simulink model "Detumbling"  (R2024b)
settings: Solver=ode4  StartTime=0.0  StopTime=2000  FixedStep=0.1  RelTol=1e-3
values from neighbouring files (symbols this model uses):
  A = A + DCM_out_slew(:,:,jj)    [sadcode.m]
  a = 6899750    [sadcode.m]
  Area_vect = [3;3;3;3;1;1;1;1;1;1]    [sadcode.m]
  C_d = 2.2    [sadcode.m]
  e = 0.0005895    [sadcode.m]
  G = 6.67e-11    [sadcode.m]
  g = [g1_0 g2_0 g3_0 g4_0 g5_0 g6_0 g7_0 g8_0 g9_0 g10_0  g11_0  g12_0  g13_0 ... (first row only)    [IGRF13.m]
  h = [h1_0 h2_0 h3_0 h4_0 h5_0 h6_0 h7_0 h8_0 h9_0 h10_0  h11_0  h12_0  h13_0 ... (first row only)    [IGRF13.m]
  I = diag([Ix,Iy,Iz])    [sadcode.m]
  i = deg2rad(5.0097)    [sadcode.m]
  Ix = 4.208e11*10^(-3-6)    (= 420.8)    [sadcode.m]
  Iy = 4.922e12*10^(-3-6)    (= 4922)    [sadcode.m]
  Iz = 4.399e12*10^(-3-6)    (= 4399)    [sadcode.m]
  J_b = [1 ; 18 ; 5]    [sadcode.m]
  k_det = 110    [sadcode.m]
  M = 5.97219e24    (= 5.97219e+24)    [sadcode.m]
  Mount = [0 0 1 0 1 0]    [sadcode.m]
  mu = G*M    (= 398345073000000)    [sadcode.m]
  n = sqrt(mu/a^3)    [sadcode.m]
  N_b = [0,0,+1; 0,0,-1; 0,0,1; 0,0,-1;1,0,0 ; -1,0,0; 0,1,0; 0,-1,0; 0,0,1; 0,0,-1]    [sadcode.m]
  n_face = length(rho_s)    [sadcode.m]
  p = a * (1 - e^2)    (= 6899747.60227)    [sadcode.m]
  q = abs(q(:,1))    [sadcode.m]
  R_f = [2.5,0,0; 2.5,0,0; -2.5,0,0; -2.5,0,0; 1,0,0; -1,0,0; 0,1,0; 0,-1,0; 0,0,1; 0,0,-1]    [sadcode.m]
  R_sun = 149597870700    [sadcode.m]
  rho = 3.13e-13    [sadcode.m]
  theta0 = theta0_slew(jj)    [sadcode.m]
  w0x = w_out_slew(1,jj)    [sadcode.m]
  w0y = w_out_slew(2,jj)    [sadcode.m]
  w0z = w_out_slew(3,jj)    [sadcode.m]
  w_earth = 2*pi/(24*3600)    (= 7.27220521664e-05)    [sadcode.m]
undefined symbols (not defined in the file or in its folder): DiscIntNeverNeededParam
libraries: matrix_library x6, simulink x5
settings Model: Creator=andre  LastModifiedBy=andre
settings OptimizationCC: ReuseModelBlockBuffer=off
settings RTWCC: GPUComputeCapability=3.5

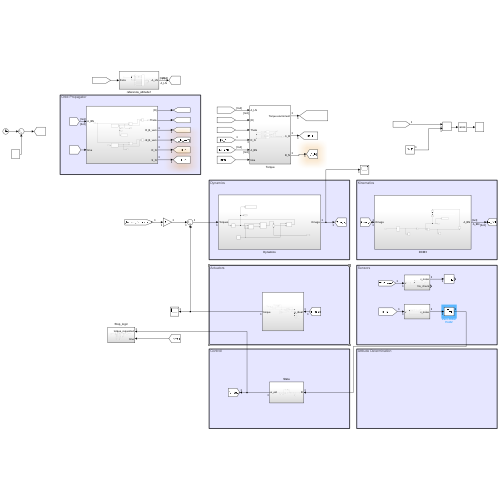
[thumbnail: Simulink's stored preview of the top-level diagram]
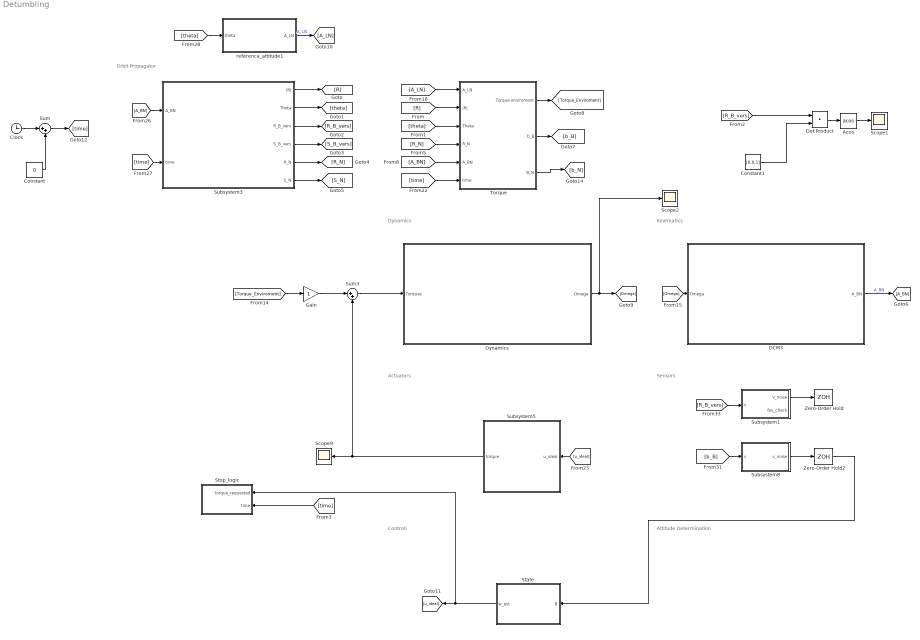
== system Detumbling ==
  note: Orbit Propagator
  note: Dynamics
  note: Kinematics
  note: Sensors
  note: Attitude Determination
  note: Controll
  note: Actuators
  Acos : Trigonometry  Operator=acos
  Clock : Clock
  Constant : Constant  Value=0
  Constant1 : Constant  Value=[0,0,1]
  DCM3 : Subsystem
  Dot Product : DotProduct  OutDataTypeStr=Inherit: Inherit via internal rule
  Dynamics : Subsystem
  Gain : Gain
  Scope1 : Scope
  Scope2 : Scope
  Scope9 : Scope
  State : Subsystem
  Stop_logic : Subsystem
  Subsystem1 : Subsystem
  Subsystem3 : Subsystem
  Subsystem5 : Subsystem
  Subsystem8 : Subsystem
  Sum : Sum  Inputs=|++
  Sum3 : Sum  Inputs=|++
  Torque : Subsystem
  Zero-Order Hold : ZeroOrderHold
  Zero-Order Hold2 : ZeroOrderHold  SampleTime=0.1
  referenca_attitude1 : Subsystem
  wires:
  Sum3/1 -> Dynamics/1(Torques)
  Subsystem5/1(torque) -> Scope9/1, Sum3/2
  Subsystem3/2(Theta) -> [theta]
  Subsystem3/3(R_B_vers) -> [R_B_vers]
  Subsystem3/4(S_B_vers) -> [S_B_vers]
  Subsystem3/5(R_N) -> [R_N]
  Subsystem3/6(S_N) -> [S_N]
  DCM3/1(A_BN) -> [A_BN]  "A_BN"
  [Torque_Enviroment] -> Gain/1
  Dynamics/1(Omega) -> Scope2/1, [Omega]
  [Omega] -> DCM3/1(Omega)
  referenca_attitude1/1(A_LN) -> [A_LN]  "A_LN"
  [theta] -> referenca_attitude1/1(theta)
  [u_ideal] -> Subsystem5/1(u_ideal)
  Subsystem3/1(|R|) -> [R]
  Clock/1 -> Sum/1
  Constant/1 -> Sum/2
  Sum/1 -> [time]
  [A_BN] -> Subsystem3/1(A_BN)
  [time] -> Subsystem3/2(time)
  State/1(w_est) -> Stop_logic/1(torque_requested), [u_ideal]
  [b_B] -> Subsystem8/1(v)
  [R_B_vers] -> Subsystem1/1(v)
  Subsystem8/1(v_noise) -> Zero-Order Hold2/1
  Subsystem1/1(v_noise) -> Zero-Order Hold/1
  Zero-Order Hold2/1 -> State/1(B)
  Gain/1 -> Sum3/1
  [R_B_vers] -> Dot Product/1
  Constant1/1 -> Dot Product/2
  Dot Product/1 -> Acos/1
  Acos/1 -> Scope1/1
  [time] -> Stop_logic/2(time)
  [A_LN] -> Torque/1(A_LN)
  [R_N] -> Torque/4(R_N)
  [A_BN] -> Torque/5(A_BN)
  [time] -> Torque/6(time)
  [R] -> Torque/2(|R|)
  [theta] -> Torque/3(Theta)
  Torque/1(Torque enviroment) -> [Torque_Enviroment]
  Torque/3(B_N) -> [b_N]
  Torque/2(b_B) -> [b_B]

== system Detumbling/DCM3 ==
  note: YOU CAN ORTHORNORMALIZE MORE TIMES
  Omega : Inport
  Gain : Gain  Gain=-1
  Integrator3 : Integrator  InitialCondition=A
  ORTHONORMALIZE1 : Subsystem
  ORTHONORMALIZE3 : Subsystem
  Product3 : Product  Multiplication=Matrix(*)
  Scope : Scope
  Scope2 : Scope
  To Workspace1 : ToWorkspace  VariableName=real_DCM_det  SampleTime=-1
  w->w^ : Subsystem
  A_BN : Outport
  wires:
  Gain/1 -> Product3/1
  Omega/1 -> w->w^/1(In1)
  w->w^/1(Out1) -> Gain/1, Scope/1
  Product3/1 -> Integrator3/1, Scope2/1
  Integrator3/1 -> ORTHONORMALIZE1/1(In1)
  ORTHONORMALIZE1/1(u) -> ORTHONORMALIZE3/1(In1)
  ORTHONORMALIZE3/1(u) -> To Workspace1/1, A_BN/1, Product3/2

== system Detumbling/Dynamics ==
  Torques : Inport
  Constant : Constant  Value=I
  Cross Product : matrix_library/Cross Product
  Integrator : Integrator  InitialCondition=[w0x;w0y;w0z]
  Matrix Multiply2 : Product  Inputs=/*  Multiplication=Matrix(*)
  Matrix Multiply3 : Product  Inputs=**  Multiplication=Matrix(*)
  Sum1 : Sum  Inputs=-+
  To Workspace : ToWorkspace  VariableName=w_out_det  SampleTime=-1
  Omega : Outport
  wires:
  Matrix Multiply2/1 -> Integrator/1
  Matrix Multiply3/1 -> Cross Product/2
  Cross Product/1 -> Sum1/1
  Constant/1 -> Matrix Multiply2/1, Matrix Multiply3/1
  Torques/1 -> Sum1/2
  Integrator/1 -> Cross Product/1, Matrix Multiply3/2, To Workspace/1, Omega/1
  Sum1/1 -> Matrix Multiply2/2

== system Detumbling/State ==
  B : Inport
  Cross Product : matrix_library/Cross Product
  Discrete Derivative : simulink/Discrete/Discrete Derivative  gainval=1.0  ICPrevScaledInput=0.0  OutMin=[]  OutMax=[]  OutDataType=fixdt(1, 16)  OutScaling=2^-10  DoSatur=off
  Gain : Gain  Gain=k_det
  Product : Product  Inputs=/*
  Scope : Scope
  Square : Math  Operator=square
  normalize2 : Subsystem
  w_est : Outport
  wires:
  Discrete Derivative/1 -> Cross Product/2
  Cross Product/1 -> Product/2
  normalize2/2(norm) -> Square/1
  Square/1 -> Product/1
  Product/1 -> Gain/1
  B/1 -> Discrete Derivative/1, normalize2/1(vector), Cross Product/1
  Gain/1 -> Scope/1, w_est/1

== system Detumbling/Stop_logic ==
  torque_requested : Inport
  time : Inport  Port=2
  AND : Logic  IconShape=distinctive  AllPortsSameDT=off  OutDataTypeStr=boolean
  Constant2 : Constant  Value=2.5
  Constant3 : Constant  Value=100
  Integrator : Integrator
  Relational Operator : RelationalOperator  Operator=<=  OutDataTypeStr=boolean  RndMeth=Simplest  InputSameDT=off
  Relational Operator1 : RelationalOperator  Operator=>  OutDataTypeStr=boolean  RndMeth=Simplest  InputSameDT=off
  Scope2 : Scope
  Scope3 : Scope
  Stop Simulation : Stop
  Sum1 : Sum  Inputs=|+-
  Transport Delay : TransportDelay  DelayTime=10
  normalize2 : Subsystem
  wires:
  Relational Operator1/1 -> AND/1
  time/1 -> Relational Operator1/1
  AND/1 -> Stop Simulation/1
  Sum1/1 -> Scope2/1, Relational Operator/1
  Constant2/1 -> Relational Operator/2
  Constant3/1 -> Relational Operator1/2
  Integrator/1 -> Transport Delay/1, Sum1/1
  Relational Operator/1 -> Scope3/1, AND/2
  Transport Delay/1 -> Sum1/2
  normalize2/2(norm) -> Integrator/1
  torque_requested/1 -> normalize2/1(vector)

== system Detumbling/Subsystem1 ==
  v : Inport
  Constant : Constant  Value=[0,0,1]
  Cross Product : matrix_library/Cross Product
  FOV_check : Subsystem
  Product : Product
  Scope : Scope
  Scope1 : Scope
  Subsystem : Subsystem
  Subsystem3 : Subsystem
  normalize1 : Subsystem
  v_noise : Outport
  fov_check : Outport  Port=2
  wires:
  Product/1 -> v_noise/1, Scope1/1
  Cross Product/1 -> Subsystem/2(n)
  Constant/1 -> Cross Product/2
  Subsystem/1(Out1) -> Scope/1, Subsystem3/1(v)
  FOV_check/1(v_checked) -> Subsystem3/2(n), Subsystem/1(v), Cross Product/1
  FOV_check/2(fov_check) -> fov_check/1
  v/1 -> normalize1/1(vector)
  normalize1/1(vers) -> FOV_check/1(R_B_vers)
  Subsystem3/1(v_noise) -> Product/1
  normalize1/2(norm) -> Product/2

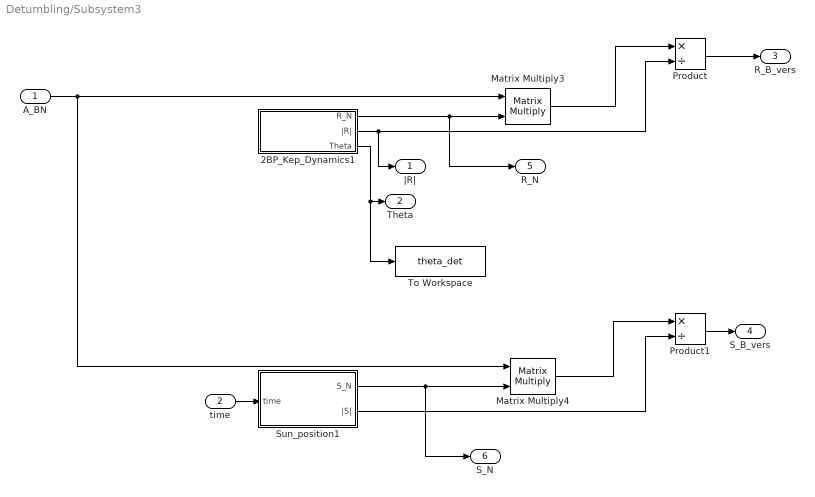
== system Detumbling/Subsystem3 ==
  A_BN : Inport
  time : Inport  Port=2
  2BP_Kep_Dynamics1 : Subsystem
  Matrix Multiply3 : Product  Multiplication=Matrix(*)
  Matrix Multiply4 : Product  Multiplication=Matrix(*)
  Product : Product  Inputs=*/
  Product1 : Product  Inputs=*/
  Sun_position1 : Subsystem
  To Workspace : ToWorkspace  VariableName=theta_det  SampleTime=-1
  |R| : Outport
  Theta : Outport  Port=2
  R_B_vers : Outport  Port=3
  S_B_vers : Outport  Port=4
  R_N : Outport  Port=5
  S_N : Outport  Port=6
  wires:
  A_BN/1 -> Matrix Multiply3/1, Matrix Multiply4/1
  2BP_Kep_Dynamics1/2(|R|) -> Product/2, |R|/1
  Matrix Multiply3/1 -> Product/1
  Matrix Multiply4/1 -> Product1/1
  2BP_Kep_Dynamics1/1(R_N) -> Matrix Multiply3/2, R_N/1
  Sun_position1/2(|S|) -> Product1/2
  Sun_position1/1(S_N) -> Matrix Multiply4/2, S_N/1
  2BP_Kep_Dynamics1/3(Theta) -> To Workspace/1, Theta/1
  Product/1 -> R_B_vers/1
  Product1/1 -> S_B_vers/1
  time/1 -> Sun_position1/1(time)

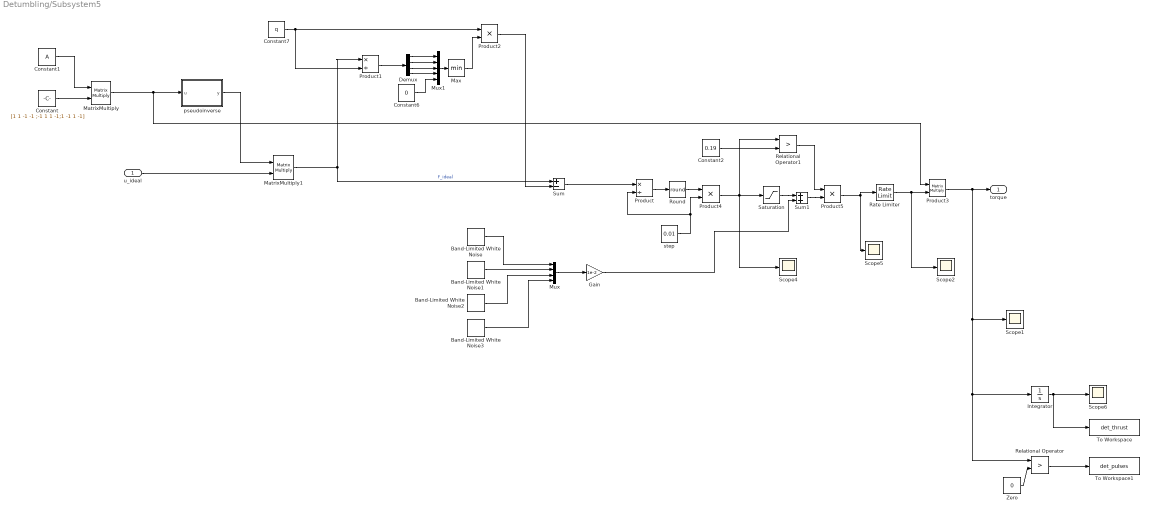
== system Detumbling/Subsystem5 ==
  u_ideal : Inport
  Band-Limited White Noise{,1..3} (4 alike) : simulink/Sources/Band-Limited White Noise  Cov=[1]  Ts=0.1  seed=[23341]
  Constant : Constant  Value=[1 1 -1 -1 ;-1 1 1 -1;1 -1 1 -1]
  Constant1 : Constant  Value=A
  Constant2 : Constant  Value=0.19
  Constant6 : Constant  Value=0
  Constant7 : Constant  Value=q
  Demux : Demux
  Gain : Gain  Gain=1e-2
  Integrator : Integrator
  MatrixMultiply : Product  Multiplication=Matrix(*)
  MatrixMultiply1 : Product  Multiplication=Matrix(*)
  Max : MinMax
  Mux : Mux
  Mux1 : Mux  Inputs=5
  Product : Product  Inputs=*/
  Product1 : Product  Inputs=*/
  Product2 : Product
  Product3 : Product  Multiplication=Matrix(*)
  Product4 : Product  Inputs=**
  Product5 : Product
  Rate Limiter : RateLimiter  RisingSlewLimit=0.5  FallingSlewLimit=-0.5  SampleTimeMode=inherited
  Relational Operator : RelationalOperator  Operator=>  OutDataTypeStr=boolean  RndMeth=Simplest  InputSameDT=off
  Relational Operator1 : RelationalOperator  Operator=>  OutDataTypeStr=boolean  RndMeth=Simplest  InputSameDT=off
  Round : Rounding  Operator=round
  Saturation : Saturate  UpperLimit=1.13  LowerLimit=0.19
  Scope{1..2,4..6} (5 alike) : Scope
  Sum : Sum  Inputs=+-
  Sum1 : Sum
  To Workspace : ToWorkspace  VariableName=det_thrust  SampleTime=-1
  To Workspace1 : ToWorkspace  VariableName=det_pulses  SampleTime=-1
  Zero : Constant  Value=0  OutDataTypeStr=Inherit: Inherit via back propagation
  pseudoinverse : MATLAB Function  TreatAsAtomicUnit=on
  step : Constant  Value=0.01
  torque : Outport
  wires:
  Band-Limited White Noise1/1 -> Mux/2
  Rate Limiter/1 -> Scope2/1, Product3/2
  Band-Limited White Noise2/1 -> Mux/3
  MatrixMultiply1/1 -> Sum/1, Product1/1  "F_ideal"
  Constant1/1 -> MatrixMultiply/1
  Mux/1 -> Gain/1
  Constant/1 -> MatrixMultiply/2
  Band-Limited White Noise/1 -> Mux/1
  Product1/1 -> Demux/1
  Band-Limited White Noise3/1 -> Mux/4
  Product2/1 -> Sum/2
  u_ideal/1 -> MatrixMultiply1/2
  pseudoinverse/1(y) -> MatrixMultiply1/1
  MatrixMultiply/1 -> Product3/1, pseudoinverse/1(u)
  Sum/1 -> Product/1
  Constant6/1 -> Mux1/5
  Constant7/1 -> Product1/2, Product2/1
  Demux/1 -> Mux1/1
  Demux/2 -> Mux1/2
  Demux/3 -> Mux1/3
  Demux/4 -> Mux1/4
  Mux1/1 -> Max/1
  Max/1 -> Product2/2
  Gain/1 -> Sum1/2
  Product5/1 -> Rate Limiter/1, Scope5/1
  Round/1 -> Product4/1
  step/1 -> Product4/2, Product/2
  Product/1 -> Round/1
  Product4/1 -> Scope4/1, Saturation/1, Relational Operator1/1
  Integrator/1 -> To Workspace/1, Scope6/1
  Zero/1 -> Relational Operator/2
  Relational Operator/1 -> To Workspace1/1
  Product3/1 -> Scope1/1, Integrator/1, Relational Operator/1, torque/1
  Relational Operator1/1 -> Product5/1
  Constant2/1 -> Relational Operator1/2
  Saturation/1 -> Sum1/1
  Sum1/1 -> Product5/2

== system Detumbling/Subsystem8 ==
  v : Inport
  Constant : Constant  Value=[0,0,1]
  Cross Product : matrix_library/Cross Product
  Product : Product
  Scope : Scope
  Scope1 : Scope
  Subsystem : Subsystem
  Subsystem3 : Subsystem
  normalize1 : Subsystem
  v_noise : Outport
  wires:
  Product/1 -> v_noise/1, Scope1/1
  Cross Product/1 -> Subsystem/2(n)
  normalize1/1(vers) -> Subsystem3/2(n), Subsystem/1(v), Cross Product/1
  Constant/1 -> Cross Product/2
  Subsystem/1(Out1) -> Scope/1, Subsystem3/1(v)
  v/1 -> normalize1/1(vector)
  Subsystem3/1(v_noise) -> Product/1
  normalize1/2(norm) -> Product/2

== system Detumbling/Torque ==
  A_LN : Inport
  |R| : Inport  Port=2
  Theta : Inport  Port=3
  R_N : Inport  Port=4
  A_BN : Inport  Port=5
  time : Inport  Port=6
  DRAG_Torque : Subsystem
  GG_Torque : Subsystem
  MAG_Torque : Subsystem
      settings: PortSchema="{\"entries\":[{\"content\":{\"sides\":[{\"content\":{\"connectorIds\":[\"In1\",\"In2\"]},\"type\":\"ConnectorPlacement.EquallySpacedRectSide\",\"uuid\":\"c54f6d6b-6c64-41b4-9c4b-666110e71804\"},{\"content\":{\"connectorIds\":[\"Out1\",\"Out2\",\"Out3\"],\"side\":\"RIGHT\"},\"type\":\"ConnectorPlacement.EquallySpacedRectSide\",\"uuid\":\"b119c4d3-4afb-4dc4-a90a-1aa1f0569df9\"},{\"content\":{\"side\":\"TOP\"},\"type\":\"ConnectorPlacement.EquallySpacedRectSide\",\"uuid\":\"da830b3a-87b4-4a36-90f7-6cd3013fb920\"},{\"content\":{\"connectorIds\":[\"In3\"],\"side\":\"BOTTOM\"},\"type\":\"ConnectorPlacement.EquallySpacedRectSide\",\"uuid\":\"c632635c-67f5-47aa-a2ed-3b005f31cd37\"}]},\"type\":\"ConnectorPlacement.EquallySpacedConnector\",\"uuid\":\"fdb04bfd-e1a8-4c42-a1d7-57e7f291fe41\"}],\"packageUris\":[\"http://schema.mathworks.com/mf0/Connector/R2020b\"],\"version\":\"1.0\"}"
  Scope : Scope
  Scope1 : Scope
  Sum : Sum  Inputs=+++
  Torque enviroment : Outport
  b_B : Outport  Port=2
  B_N : Outport  Port=3
  wires:
  |R|/1 -> GG_Torque/2(|R|)
  Theta/1 -> DRAG_Torque/2(Theta)
  A_BN/1 -> GG_Torque/3(A_BN), MAG_Torque/1(A_BN), DRAG_Torque/3(A_BN)
  A_LN/1 -> GG_Torque/1(A_LN)
  R_N/1 -> DRAG_Torque/1(R_N), MAG_Torque/2(R_N)
  GG_Torque/1(GG_Torque) -> Sum/1, Scope1/1
  MAG_Torque/1(MAG_Torque) -> Scope/1, Sum/2
  MAG_Torque/2(Out1) -> b_B/1
  Sum/1 -> Torque enviroment/1
  time/1 -> MAG_Torque/3(t)
  DRAG_Torque/1(DRAG_Torque) -> Sum/3
  MAG_Torque/3(B_N) -> B_N/1

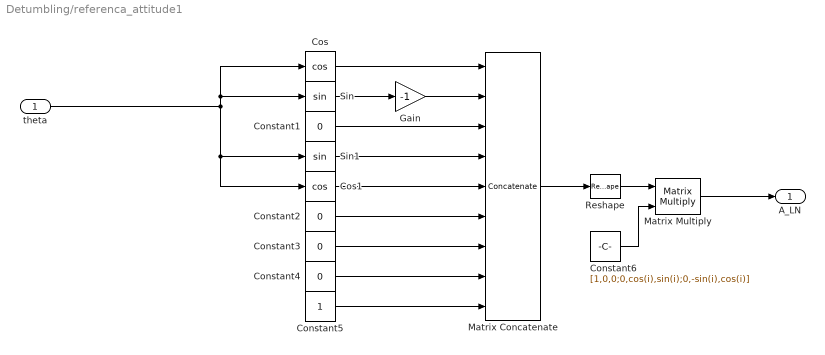
== system Detumbling/referenca_attitude1 ==
  theta : Inport
  Constant{1..4} (4 alike) : Constant  Value=0
  Constant5 : Constant
  Constant6 : Constant  Value=[1,0,0;0,cos(i),sin(i);0,-sin(i),cos(i)]
  Cos : Trigonometry  Operator=cos
  Cos1 : Trigonometry  Operator=cos
  Gain : Gain  Gain=-1
  Matrix Concatenate : Concatenate  NumInputs=9  ConcatenateDimension=2
  Matrix Multiply : Product  Multiplication=Matrix(*)
  Reshape : Reshape  OutputDimensionality=Customize  OutputDimensions=[3,3]
  Sin : Trigonometry
  Sin1 : Trigonometry
  A_LN : Outport
  wires:
  Cos/1 -> Matrix Concatenate/1
  Gain/1 -> Matrix Concatenate/2
  Sin/1 -> Gain/1
  Constant1/1 -> Matrix Concatenate/3
  Sin1/1 -> Matrix Concatenate/4
  Cos1/1 -> Matrix Concatenate/5
  Constant2/1 -> Matrix Concatenate/6
  Constant5/1 -> Matrix Concatenate/9
  Constant4/1 -> Matrix Concatenate/8
  Constant3/1 -> Matrix Concatenate/7
  theta/1 -> Cos/1, Sin/1, Cos1/1, Sin1/1
  Reshape/1 -> Matrix Multiply/1
  Matrix Concatenate/1 -> Reshape/1
  Matrix Multiply/1 -> A_LN/1
  Constant6/1 -> Matrix Multiply/2

== system Detumbling/DCM3/ORTHONORMALIZE1 ==
  In1 : Inport
  Gain : Gain  Gain=1.5
  Gain1 : Gain  Gain=-0.5
  Product : Product  Multiplication=Matrix(*)
  Product1 : Product  Multiplication=Matrix(*)
  Sum : Sum  Inputs=|++
  Transpose : Math  Operator=transpose
  u : Outport
  wires:
  Sum/1 -> u/1
  Gain1/1 -> Sum/2
  Gain/1 -> Sum/1
  Product1/1 -> Gain1/1
  Product/1 -> Product1/1
  Transpose/1 -> Product/2
  In1/1 -> Gain/1, Product/1, Transpose/1, Product1/2

== system Detumbling/DCM3/ORTHONORMALIZE3 ==
  In1 : Inport
  Gain : Gain  Gain=1.5
  Gain1 : Gain  Gain=-0.5
  Product : Product  Multiplication=Matrix(*)
  Product1 : Product  Multiplication=Matrix(*)
  Sum : Sum  Inputs=|++
  Transpose : Math  Operator=transpose
  u : Outport
  wires:
  Sum/1 -> u/1
  Gain1/1 -> Sum/2
  Gain/1 -> Sum/1
  Product1/1 -> Gain1/1
  Product/1 -> Product1/1
  Transpose/1 -> Product/2
  In1/1 -> Gain/1, Transpose/1, Product1/2, Product/1

== system Detumbling/DCM3/w->w^ ==
  In1 : Inport
  Constant1 : Constant  Value=0
  Demux : Demux  Outputs=3
  Gain{,1,3..4} (4 alike) : Gain  Gain=-1
  Matrix Concatenate : Concatenate  NumInputs=9  ConcatenateDimension=2
  Reshape : Reshape  OutputDimensionality=Customize  OutputDimensions=[3,3]
  Out1 : Outport
  wires:
  Reshape/1 -> Out1/1
  In1/1 -> Demux/1
  Gain3/1 -> Matrix Concatenate/6
  Demux/3 -> Matrix Concatenate/4, Gain/1
  Demux/2 -> Matrix Concatenate/3, Gain4/1
  Gain/1 -> Matrix Concatenate/2
  Demux/1 -> Matrix Concatenate/8, Gain3/1
  Gain4/1 -> Matrix Concatenate/7
  Matrix Concatenate/1 -> Gain1/1
  Constant1/1 -> Matrix Concatenate/9, Matrix Concatenate/1, Matrix Concatenate/5
  Gain1/1 -> Reshape/1

== system Detumbling/State/normalize2 ==
  vector : Inport
  Demux : Demux  Outputs=3
  Product : Product  Inputs=*/
  Square : Math  Operator=square
  Square Root : Sqrt
  Square1 : Math  Operator=square
  Square2 : Math  Operator=square
  Sum : Sum  Inputs=+++
  vers : Outport
  norm : Outport  Port=2
  wires:
  Square Root/1 -> norm/1, Product/2
  Demux/3 -> Square2/1
  Square2/1 -> Sum/3
  Square/1 -> Sum/1
  Square1/1 -> Sum/2
  Demux/1 -> Square/1
  Sum/1 -> Square Root/1
  vector/1 -> Product/1, Demux/1
  Demux/2 -> Square1/1
  Product/1 -> vers/1

== system Detumbling/Stop_logic/normalize2 ==
  vector : Inport
  Demux : Demux  Outputs=3
  Product : Product  Inputs=*/
  Square : Math  Operator=square
  Square Root : Sqrt
  Square1 : Math  Operator=square
  Square2 : Math  Operator=square
  Sum : Sum  Inputs=+++
  vers : Outport
  norm : Outport  Port=2
  wires:
  Square Root/1 -> norm/1, Product/2
  Demux/3 -> Square2/1
  Square2/1 -> Sum/3
  Square/1 -> Sum/1
  Square1/1 -> Sum/2
  Demux/1 -> Square/1
  Sum/1 -> Square Root/1
  vector/1 -> Product/1, Demux/1
  Demux/2 -> Square1/1
  Product/1 -> vers/1

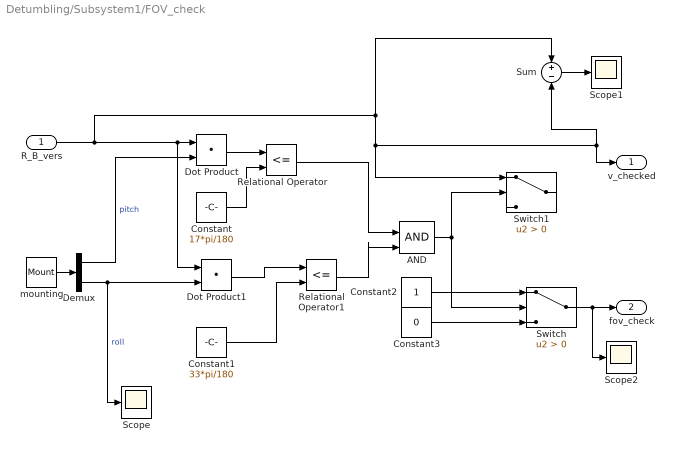
== system Detumbling/Subsystem1/FOV_check ==
  R_B_vers : Inport
  AND : Logic  IconShape=distinctive  AllPortsSameDT=off  OutDataTypeStr=boolean
  Constant : Constant  Value=17*pi/180
  Constant1 : Constant  Value=33*pi/180
  Constant2 : Constant
  Constant3 : Constant  Value=0
  Demux : Demux  Outputs=2
  Dot Product : DotProduct  OutDataTypeStr=Inherit: Inherit via internal rule
  Dot Product1 : DotProduct  OutDataTypeStr=Inherit: Inherit via internal rule
  Relational Operator : RelationalOperator  Operator=<=  OutDataTypeStr=boolean  RndMeth=Simplest  InputSameDT=off
  Relational Operator1 : RelationalOperator  Operator=<=  OutDataTypeStr=boolean  RndMeth=Simplest  InputSameDT=off
  Scope : Scope
  Scope1 : Scope
  Scope2 : Scope
  Sum : Sum  Inputs=+-
  Switch : Switch  Criteria=u2 > Threshold  SaturateOnIntegerOverflow=off  InputSameDT=off
  Switch1 : Switch  Criteria=u2 > Threshold  SaturateOnIntegerOverflow=off  InputSameDT=off
  mounting : Constant  Value=Mount
  v_checked : Outport
  fov_check : Outport  Port=2
  wires:
  Sum/1 -> Scope1/1
  mounting/1 -> Demux/1
  Demux/1 -> Dot Product/2  "pitch"
  Demux/2 -> Scope/1, Dot Product1/2  "roll"
  Switch/1 -> fov_check/1, Scope2/1
  Dot Product/1 -> Relational Operator/1
  Dot Product1/1 -> Relational Operator1/1
  AND/1 -> Switch1/2, Switch/2
  Relational Operator/1 -> AND/1
  Relational Operator1/1 -> AND/2
  Constant/1 -> Relational Operator/2
  Constant1/1 -> Relational Operator1/2
  R_B_vers/1 -> v_checked/1, Sum/2, Switch1/1, Sum/1, Dot Product1/1, Dot Product/1
  Constant2/1 -> Switch/1
  Constant3/1 -> Switch/3

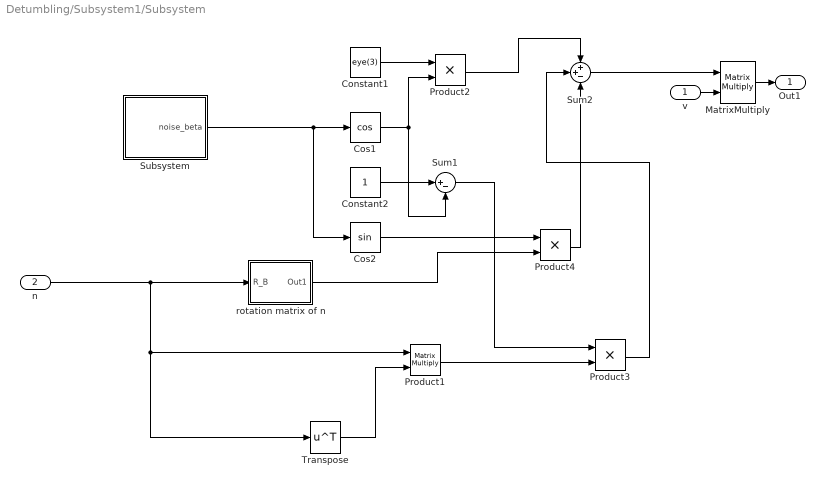
== system Detumbling/Subsystem1/Subsystem ==
  v : Inport
  n : Inport  Port=2
  Constant1 : Constant  Value=eye(3)
  Constant2 : Constant
  Cos1 : Trigonometry  Operator=cos
  Cos2 : Trigonometry
  MatrixMultiply : Product  Multiplication=Matrix(*)
  Product1 : Product  Multiplication=Matrix(*)
  Product2 : Product
  Product3 : Product
  Product4 : Product
  Subsystem : Subsystem
  Sum1 : Sum  Inputs=|+-
  Sum2 : Sum  Inputs=++-
  Transpose : Math  Operator=transpose
  rotation matrix of n : Subsystem
  Out1 : Outport
  wires:
  v/1 -> MatrixMultiply/2
  n/1 -> rotation matrix of n/1(R_B), Product1/1, Transpose/1
  Cos1/1 -> Product2/2, Sum1/2
  Sum1/1 -> Product3/1
  Product4/1 -> Sum2/3
  Product2/1 -> Sum2/1
  Cos2/1 -> Product4/1
  Subsystem/1(noise_beta) -> Cos1/1, Cos2/1
  Product1/1 -> Product3/2
  Product3/1 -> Sum2/2
  Constant1/1 -> Product2/1
  Sum2/1 -> MatrixMultiply/1
  Constant2/1 -> Sum1/1
  MatrixMultiply/1 -> Out1/1
  rotation matrix of n/1(Out1) -> Product4/2
  Transpose/1 -> Product1/2

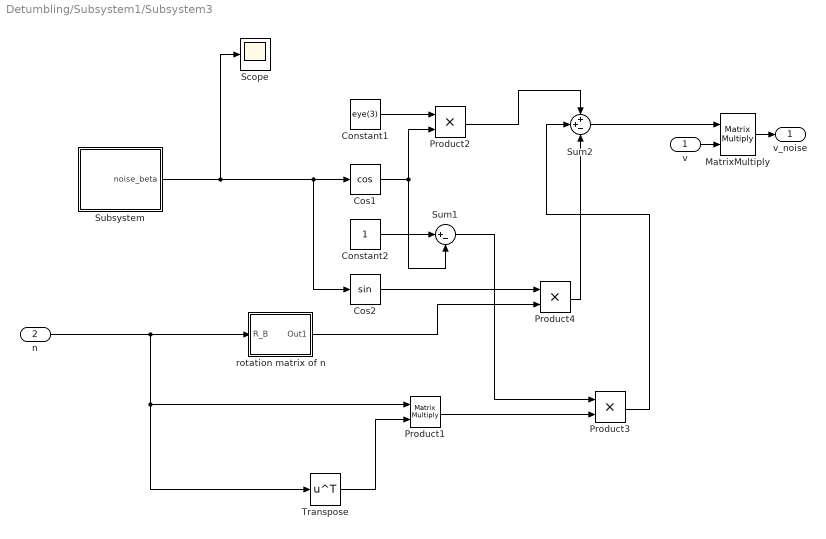
== system Detumbling/Subsystem1/Subsystem3 ==
  v : Inport
  n : Inport  Port=2
  Constant1 : Constant  Value=eye(3)
  Constant2 : Constant
  Cos1 : Trigonometry  Operator=cos
  Cos2 : Trigonometry
  MatrixMultiply : Product  Multiplication=Matrix(*)
  Product1 : Product  Multiplication=Matrix(*)
  Product2 : Product
  Product3 : Product
  Product4 : Product
  Scope : Scope
  Subsystem : Subsystem
  Sum1 : Sum  Inputs=|+-
  Sum2 : Sum  Inputs=++-
  Transpose : Math  Operator=transpose
  rotation matrix of n : Subsystem
  v_noise : Outport
  wires:
  Transpose/1 -> Product1/2
  rotation matrix of n/1(Out1) -> Product4/2
  MatrixMultiply/1 -> v_noise/1
  Constant2/1 -> Sum1/1
  Sum2/1 -> MatrixMultiply/1
  Constant1/1 -> Product2/1
  Product3/1 -> Sum2/2
  Product1/1 -> Product3/2
  Subsystem/1(noise_beta) -> Scope/1, Cos2/1, Cos1/1
  Cos2/1 -> Product4/1
  Product2/1 -> Sum2/1
  Product4/1 -> Sum2/3
  Sum1/1 -> Product3/1
  Cos1/1 -> Sum1/2, Product2/2
  n/1 -> Transpose/1, Product1/1, rotation matrix of n/1(R_B)
  v/1 -> MatrixMultiply/2

== system Detumbling/Subsystem1/normalize1 ==
  vector : Inport
  Demux : Demux  Outputs=3
  Product : Product  Inputs=*/
  Square : Math  Operator=square
  Square Root : Sqrt
  Square1 : Math  Operator=square
  Square2 : Math  Operator=square
  Sum : Sum  Inputs=+++
  vers : Outport
  norm : Outport  Port=2
  wires:
  Square Root/1 -> norm/1, Product/2
  Demux/3 -> Square2/1
  Square2/1 -> Sum/3
  Square/1 -> Sum/1
  Square1/1 -> Sum/2
  Demux/1 -> Square/1
  Sum/1 -> Square Root/1
  vector/1 -> Product/1, Demux/1
  Demux/2 -> Square1/1
  Product/1 -> vers/1

== system Detumbling/Subsystem3/2BP_Kep_Dynamics1 ==
  Constant1 : Constant
  Constant2 : Constant  Value=e
  R_norn : Subsystem
  R_vector_calc : Subsystem
  theta_integration : Subsystem
  R_N : Outport
  |R| : Outport  Port=2
  Theta : Outport  Port=3
  wires:
  Constant2/1 -> R_norn/2(e), theta_integration/2(e)
  Constant1/1 -> theta_integration/1(In1)
  theta_integration/1(Theta) -> Theta/1, R_vector_calc/1(theta)
  R_norn/1(|R|) -> |R|/1, R_vector_calc/2(|R|)
  theta_integration/2(ecos(theta)) -> R_norn/1(ecos(theta))
  R_vector_calc/1(R_N) -> R_N/1

== system Detumbling/Subsystem3/Sun_position1 ==
  time : Inport
  Constant : Constant  Value=R_sun
  Constant1 : Constant  Value=2*pi/(3600*24*365)
  Cos : Trigonometry  Operator=cos
  Mux : Mux  Inputs=3
  Product{,1..3} (4 alike) : Product
  Sin : Trigonometry
  Sin1 : Trigonometry
  cos : Constant  Value=cos(23.45/180*pi)
  sin : Constant  Value=sin(23.45/180*pi)
  S_N : Outport
  |S| : Outport  Port=2
  wires:
  Sin1/1 -> Product2/1
  Cos/1 -> Mux/1
  Product1/1 -> Mux/2
  cos/1 -> Product1/2
  sin/1 -> Product2/2
  Product/1 -> Sin1/1, Sin/1, Cos/1
  Sin/1 -> Product1/1
  Product2/1 -> Mux/3
  Mux/1 -> Product3/2
  Constant1/1 -> Product/1
  Product3/1 -> S_N/1
  Constant/1 -> |S|/1, Product3/1
  time/1 -> Product/2

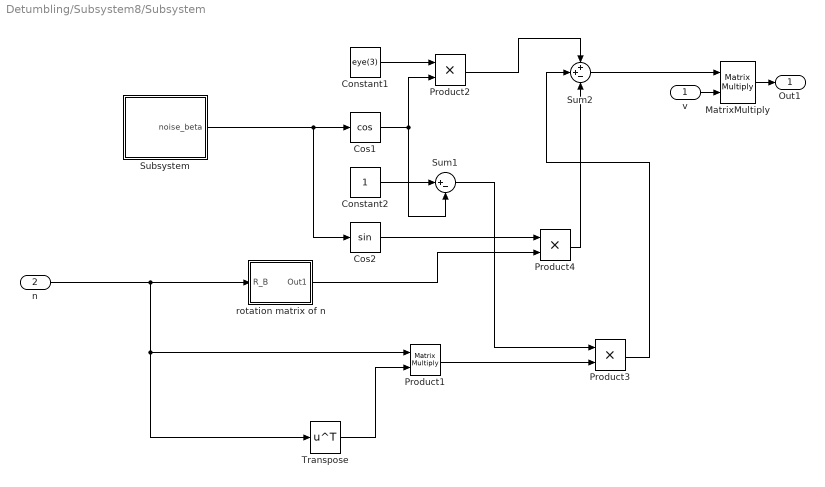
== system Detumbling/Subsystem8/Subsystem ==
  v : Inport
  n : Inport  Port=2
  Constant1 : Constant  Value=eye(3)
  Constant2 : Constant
  Cos1 : Trigonometry  Operator=cos
  Cos2 : Trigonometry
  MatrixMultiply : Product  Multiplication=Matrix(*)
  Product1 : Product  Multiplication=Matrix(*)
  Product2 : Product
  Product3 : Product
  Product4 : Product
  Subsystem : Subsystem
  Sum1 : Sum  Inputs=|+-
  Sum2 : Sum  Inputs=++-
  Transpose : Math  Operator=transpose
  rotation matrix of n : Subsystem
  Out1 : Outport
  wires:
  v/1 -> MatrixMultiply/2
  n/1 -> rotation matrix of n/1(R_B), Product1/1, Transpose/1
  Cos1/1 -> Product2/2, Sum1/2
  Sum1/1 -> Product3/1
  Product4/1 -> Sum2/3
  Product2/1 -> Sum2/1
  Cos2/1 -> Product4/1
  Subsystem/1(noise_beta) -> Cos1/1, Cos2/1
  Product1/1 -> Product3/2
  Product3/1 -> Sum2/2
  Constant1/1 -> Product2/1
  Sum2/1 -> MatrixMultiply/1
  Constant2/1 -> Sum1/1
  MatrixMultiply/1 -> Out1/1
  rotation matrix of n/1(Out1) -> Product4/2
  Transpose/1 -> Product1/2

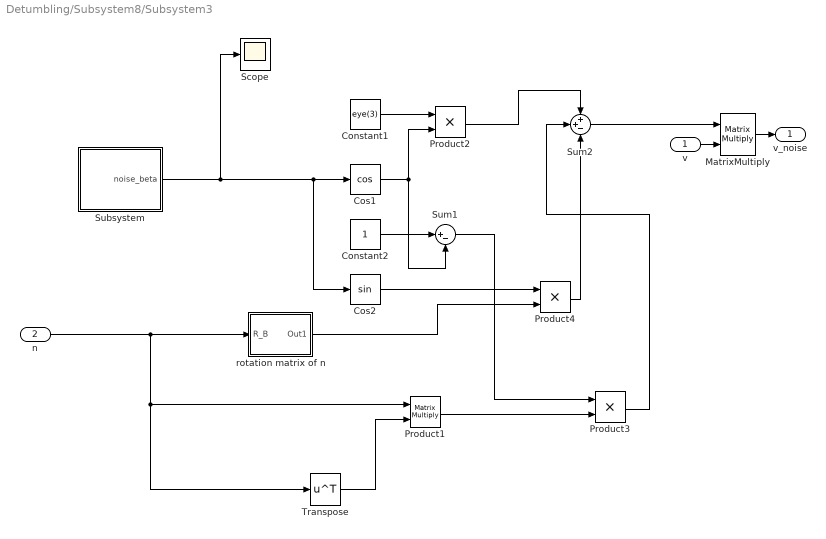
== system Detumbling/Subsystem8/Subsystem3 ==
  v : Inport
  n : Inport  Port=2
  Constant1 : Constant  Value=eye(3)
  Constant2 : Constant
  Cos1 : Trigonometry  Operator=cos
  Cos2 : Trigonometry
  MatrixMultiply : Product  Multiplication=Matrix(*)
  Product1 : Product  Multiplication=Matrix(*)
  Product2 : Product
  Product3 : Product
  Product4 : Product
  Scope : Scope
  Subsystem : Subsystem
  Sum1 : Sum  Inputs=|+-
  Sum2 : Sum  Inputs=++-
  Transpose : Math  Operator=transpose
  rotation matrix of n : Subsystem
  v_noise : Outport
  wires:
  Transpose/1 -> Product1/2
  rotation matrix of n/1(Out1) -> Product4/2
  MatrixMultiply/1 -> v_noise/1
  Constant2/1 -> Sum1/1
  Sum2/1 -> MatrixMultiply/1
  Constant1/1 -> Product2/1
  Product3/1 -> Sum2/2
  Product1/1 -> Product3/2
  Subsystem/1(noise_beta) -> Scope/1, Cos2/1, Cos1/1
  Cos2/1 -> Product4/1
  Product2/1 -> Sum2/1
  Product4/1 -> Sum2/3
  Sum1/1 -> Product3/1
  Cos1/1 -> Sum1/2, Product2/2
  n/1 -> Transpose/1, Product1/1, rotation matrix of n/1(R_B)
  v/1 -> MatrixMultiply/2

== system Detumbling/Subsystem8/normalize1 ==
  vector : Inport
  Demux : Demux  Outputs=3
  Product : Product  Inputs=*/
  Square : Math  Operator=square
  Square Root : Sqrt
  Square1 : Math  Operator=square
  Square2 : Math  Operator=square
  Sum : Sum  Inputs=+++
  vers : Outport
  norm : Outport  Port=2
  wires:
  Square Root/1 -> norm/1, Product/2
  Demux/3 -> Square2/1
  Square2/1 -> Sum/3
  Square/1 -> Sum/1
  Square1/1 -> Sum/2
  Demux/1 -> Square/1
  Sum/1 -> Square Root/1
  vector/1 -> Product/1, Demux/1
  Demux/2 -> Square1/1
  Product/1 -> vers/1

== system Detumbling/Torque/DRAG_Torque ==
  R_N : Inport
  Theta : Inport  Port=2
  A_BN : Inport  Port=3
  Constant : Constant  Value=[0,0,w_earth]
  Cross Product : matrix_library/Cross Product
  Force : Subsystem
  Scope : Scope
  Scope1 : Scope
  Sum : Subsystem
  Sum2 : Sum  Inputs=-+
  Torque : Subsystem
  V_BN : Product  Multiplication=Matrix(*)
  V_vect : Subsystem
  DRAG_Torque : Outport
  wires:
  Theta/1 -> V_vect/1(Theta)
  V_vect/1(Out1) -> Scope1/1, Sum2/2
  A_BN/1 -> V_BN/1
  Force/1(Out1) -> Torque/1(Force)
  Sum/1(Out1) -> DRAG_Torque/1, Scope/1
  Torque/1(Out1) -> Sum/1(In1)
  Constant/1 -> Cross Product/1
  R_N/1 -> Cross Product/2
  V_BN/1 -> Force/1(V_BN)
  Cross Product/1 -> Sum2/1
  Sum2/1 -> V_BN/2

== system Detumbling/Torque/GG_Torque ==
  A_LN : Inport
  |R| : Inport  Port=2
  A_BN : Inport  Port=3
  A_BL1 : Subsystem
  GG_Torque_calc : Subsystem
      settings: PortSchema="{\"entries\":[{\"content\":{\"sides\":[{\"content\":{\"connectorIds\":[]},\"type\":\"ConnectorPlacement.EquallySpacedRectSide\",\"uuid\":\"b3e24ab0-8d0b-4bc6-bdbd-4ec1f7476bbb\"},{\"content\":{\"connectorIds\":[\"Out1\"],\"side\":\"RIGHT\"},\"type\":\"ConnectorPlacement.EquallySpacedRectSide\",\"uuid\":\"8885b801-254f-4f2a-b905-f54188fcdebf\"},{\"content\":{\"connectorIds\":[\"In1\",\"In2\"],\"side\":\"TOP\"},\"type\":\"ConnectorPlacement.EquallySpacedRectSide\",\"uuid\":\"8a83708f-f116-4d47-8956-fc38ac3514b8\"}]},\"type\":\"ConnectorPlacement.EquallySpacedConnector\",\"uuid\":\"dc1ebd6b-c914-4ada-9215-47cc165cab0d\"}],\"packageUris\":[\"http://schema.mathworks.com/mf0/Connector/R2020b\"],\"version\":\"1.0\"}"
  Scope : Scope
  Subsystem : Subsystem
  GG_Torque : Outport
  wires:
  A_BL1/1(A_BL) -> Subsystem/1(A_BL)  "A_BL"
  Subsystem/1(c_vector) -> GG_Torque_calc/1(In1)
  A_LN/1 -> A_BL1/1(A_LN)
  A_BN/1 -> A_BL1/2(A_BN)
  |R|/1 -> GG_Torque_calc/2(|R|)
  GG_Torque_calc/1(GG_Torque) -> Scope/1, GG_Torque/1  "GG_Torque"

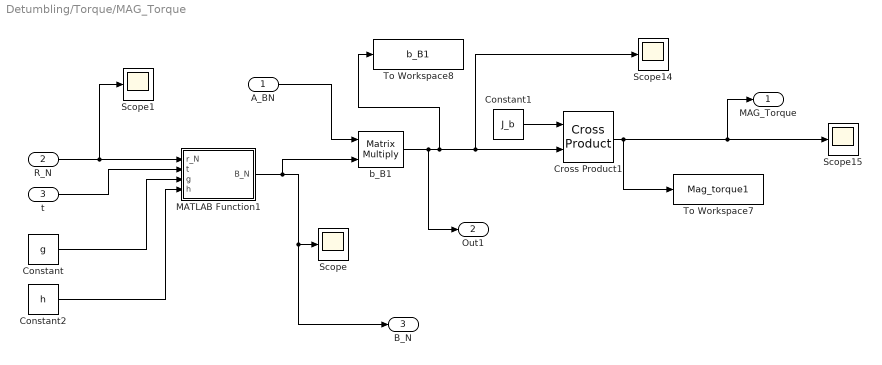
== system Detumbling/Torque/MAG_Torque ==
  A_BN : Inport
  R_N : Inport  Port=2
  t : Inport  Port=3
  Constant : Constant  Value=g
  Constant1 : Constant  Value=J_b
  Constant2 : Constant  Value=h
  Cross Product1 : matrix_library/Cross Product
  MATLAB Function1 : MATLAB Function  TreatAsAtomicUnit=on
  Scope{,1,14..15} (4 alike) : Scope
  To Workspace7 : ToWorkspace  VariableName=Mag_torque1  SampleTime=-1
  To Workspace8 : ToWorkspace  VariableName=b_B1  SampleTime=-1
  b_B1 : Product  Multiplication=Matrix(*)
  MAG_Torque : Outport
  Out1 : Outport  Port=2
  B_N : Outport  Port=3
  wires:
  A_BN/1 -> b_B1/1
  Constant1/1 -> Cross Product1/1
  b_B1/1 -> Out1/1, To Workspace8/1, Cross Product1/2, Scope14/1
  Cross Product1/1 -> To Workspace7/1, MAG_Torque/1, Scope15/1
  R_N/1 -> MATLAB Function1/1(r_N), Scope1/1
  t/1 -> MATLAB Function1/2(t)
  MATLAB Function1/1(B_N) -> B_N/1, Scope/1, b_B1/2
  Constant/1 -> MATLAB Function1/3(g)
  Constant2/1 -> MATLAB Function1/4(h)

== system Detumbling/Subsystem1/Subsystem/Subsystem ==
  Amplitude : Constant  Value=0.042/180*pi/3
  Amplitude1 : Constant  Value=0.042/180*pi/3
  Discrete-Time Integrator1 : DiscreteIntegrator  SampleTime=-1  ICPrevOutput=DiscIntNeverNeededParam  ICPrevScaledInput=DiscIntNeverNeededParam
  Product : Product
  Product7 : Product
  Random Number : RandomNumber  SampleTime=0.1
  Random Number2 : RandomNumber  SampleTime=0.1
  Scope : Scope  NumInputPorts=2
  Scope1 : Scope
  Sum : Sum
  noise_beta : Outport
  wires:
  Discrete-Time Integrator1/1 -> Sum/2, Scope/2
  Sum/1 -> noise_beta/1, Scope1/1
  Amplitude1/1 -> Product7/2
  Product7/1 -> Discrete-Time Integrator1/1
  Random Number2/1 -> Product7/1
  Random Number/1 -> Product/1
  Amplitude/1 -> Product/2
  Product/1 -> Sum/1, Scope/1

== system Detumbling/Subsystem1/Subsystem/rotation matrix of n ==
  R_B : Inport
  Constant1 : Constant  Value=0
  Demux : Demux  Outputs=3
  Gain{,1,3..4} (4 alike) : Gain  Gain=-1
  Matrix Concatenate : Concatenate  NumInputs=9  ConcatenateDimension=2
  Reshape : Reshape  OutputDimensionality=Customize  OutputDimensions=[3,3]
  Out1 : Outport
  wires:
  Gain1/1 -> Reshape/1
  Constant1/1 -> Matrix Concatenate/5, Matrix Concatenate/1, Matrix Concatenate/9
  Matrix Concatenate/1 -> Gain1/1
  Gain4/1 -> Matrix Concatenate/7
  Demux/1 -> Gain3/1, Matrix Concatenate/8
  Gain/1 -> Matrix Concatenate/2
  Demux/2 -> Gain4/1, Matrix Concatenate/3
  Demux/3 -> Gain/1, Matrix Concatenate/4
  Gain3/1 -> Matrix Concatenate/6
  R_B/1 -> Demux/1
  Reshape/1 -> Out1/1

== system Detumbling/Subsystem1/Subsystem3/Subsystem ==
  Discrete-Time Integrator1 : DiscreteIntegrator  SampleTime=-1  ICPrevOutput=DiscIntNeverNeededParam  ICPrevScaledInput=DiscIntNeverNeededParam
  Gain : Gain  Gain=1/10
  Product : Product
  Product7 : Product
  Random Number : RandomNumber  SampleTime=0.1
  Random Number2 : RandomNumber  SampleTime=0.1
  Scope : Scope  NumInputPorts=2
  Scope1 : Scope
  Scope2 : Scope
  Sum : Sum
  brown : Constant  Value=pi
  white : Constant  Value=0.042/180*pi/3
  noise_beta : Outport
  wires:
  Gain/1 -> Sum/2, Scope/2
  Discrete-Time Integrator1/1 -> Gain/1
  Sum/1 -> noise_beta/1, Scope1/1
  brown/1 -> Product7/2
  Product7/1 -> Discrete-Time Integrator1/1, Scope2/1
  Random Number2/1 -> Product7/1
  Random Number/1 -> Product/1
  white/1 -> Product/2
  Product/1 -> Sum/1, Scope/1

== system Detumbling/Subsystem1/Subsystem3/rotation matrix of n ==
  R_B : Inport
  Constant1 : Constant  Value=0
  Demux : Demux  Outputs=3
  Gain{,1,3..4} (4 alike) : Gain  Gain=-1
  Matrix Concatenate : Concatenate  NumInputs=9  ConcatenateDimension=2
  Reshape : Reshape  OutputDimensionality=Customize  OutputDimensions=[3,3]
  Out1 : Outport
  wires:
  Reshape/1 -> Out1/1
  R_B/1 -> Demux/1
  Gain3/1 -> Matrix Concatenate/6
  Demux/3 -> Matrix Concatenate/4, Gain/1
  Demux/2 -> Matrix Concatenate/3, Gain4/1
  Gain/1 -> Matrix Concatenate/2
  Demux/1 -> Matrix Concatenate/8, Gain3/1
  Gain4/1 -> Matrix Concatenate/7
  Matrix Concatenate/1 -> Gain1/1
  Constant1/1 -> Matrix Concatenate/9, Matrix Concatenate/1, Matrix Concatenate/5
  Gain1/1 -> Reshape/1

== system Detumbling/Subsystem3/2BP_Kep_Dynamics1/R_norn ==
  ecos(theta) : Inport
  e : Inport  Port=2
  Constant : Constant  Value=a
  Constant1 : Constant
  Product2 : Product  Inputs=**/
  Square2 : Math  Operator=square
  Sum2 : Sum  Inputs=|+-
  Sum3 : Sum  Inputs=|++
  |R| : Outport
  wires:
  e/1 -> Square2/1
  Constant/1 -> Product2/1
  Constant1/1 -> Sum3/2, Sum2/1
  Sum2/1 -> Product2/2
  Sum3/1 -> Product2/3
  Square2/1 -> Sum2/2
  Product2/1 -> |R|/1
  ecos(theta)/1 -> Sum3/1

== system Detumbling/Subsystem3/2BP_Kep_Dynamics1/R_vector_calc ==
  theta : Inport
  |R| : Inport  Port=2
  Constant5 : Constant  Value=i
  Cos1 : Trigonometry  Operator=cos
  Cos2 : Trigonometry  Operator=cos
  Mux : Mux  Inputs=3
  Product3 : Product
  Product4 : Product
  Product5 : Product
  Sin : Trigonometry
  Sin1 : Trigonometry
  R_N : Outport
  wires:
  Product5/1 -> Mux/3
  theta/1 -> Cos1/1, Sin/1
  Product3/1 -> R_N/1
  Mux/1 -> Product3/1
  Sin/1 -> Product5/1, Product4/2
  |R|/1 -> Product3/2
  Constant5/1 -> Sin1/1, Cos2/1
  Cos2/1 -> Product4/1
  Sin1/1 -> Product5/2
  Product4/1 -> Mux/2
  Cos1/1 -> Mux/1

== system Detumbling/Subsystem3/2BP_Kep_Dynamics1/theta_integration ==
  In1 : Inport
  e : Inport  Port=2
  Constant3 : Constant  Value=n
  Constant4 : Constant  Value=3/2
  Cos : Trigonometry  Operator=cos
  Integrator : Integrator  InitialCondition=theta0  WrapState=on  WrappedStateUpperValue=2*pi  WrappedStateLowerValue=0
  Power : Math  Operator=pow
  Product : Product
  Product1 : Product  Inputs=**/
  Square : Math  Operator=square
  Square1 : Math  Operator=square
  Sum : Sum  Inputs=|++
  Sum1 : Sum  Inputs=|-+
  Theta : Outport
  ecos(theta) : Outport  Port=2
  wires:
  e/1 -> Product/1, Square1/1
  Integrator/1 -> Theta/1, Cos/1
  Square/1 -> Product1/2
  Cos/1 -> Product/2
  Sum/1 -> Square/1
  In1/1 -> Sum1/2, Sum/1
  Product1/1 -> Integrator/1
  Constant3/1 -> Product1/1
  Product/1 -> ecos(theta)/1, Sum/2
  Square1/1 -> Sum1/1
  Constant4/1 -> Power/2
  Sum1/1 -> Power/1
  Power/1 -> Product1/3

== system Detumbling/Subsystem8/Subsystem/Subsystem ==
  Amplitude : Constant  Value=0.042/180*pi/3
  Amplitude1 : Constant  Value=0.042/180*pi/3
  Discrete-Time Integrator1 : DiscreteIntegrator  SampleTime=-1  ICPrevOutput=DiscIntNeverNeededParam  ICPrevScaledInput=DiscIntNeverNeededParam
  Product : Product
  Product7 : Product
  Random Number : RandomNumber  SampleTime=0.1
  Random Number2 : RandomNumber  SampleTime=0.1
  Scope : Scope  NumInputPorts=2
  Scope1 : Scope
  Sum : Sum
  noise_beta : Outport
  wires:
  Discrete-Time Integrator1/1 -> Sum/2, Scope/2
  Sum/1 -> noise_beta/1, Scope1/1
  Amplitude1/1 -> Product7/2
  Product7/1 -> Discrete-Time Integrator1/1
  Random Number2/1 -> Product7/1
  Random Number/1 -> Product/1
  Amplitude/1 -> Product/2
  Product/1 -> Sum/1, Scope/1

== system Detumbling/Subsystem8/Subsystem/rotation matrix of n ==
  R_B : Inport
  Constant1 : Constant  Value=0
  Demux : Demux  Outputs=3
  Gain{,1,3..4} (4 alike) : Gain  Gain=-1
  Matrix Concatenate : Concatenate  NumInputs=9  ConcatenateDimension=2
  Reshape : Reshape  OutputDimensionality=Customize  OutputDimensions=[3,3]
  Out1 : Outport
  wires:
  Gain1/1 -> Reshape/1
  Constant1/1 -> Matrix Concatenate/5, Matrix Concatenate/1, Matrix Concatenate/9
  Matrix Concatenate/1 -> Gain1/1
  Gain4/1 -> Matrix Concatenate/7
  Demux/1 -> Gain3/1, Matrix Concatenate/8
  Gain/1 -> Matrix Concatenate/2
  Demux/2 -> Gain4/1, Matrix Concatenate/3
  Demux/3 -> Gain/1, Matrix Concatenate/4
  Gain3/1 -> Matrix Concatenate/6
  R_B/1 -> Demux/1
  Reshape/1 -> Out1/1

== system Detumbling/Subsystem8/Subsystem3/Subsystem ==
  Discrete-Time Integrator1 : DiscreteIntegrator  SampleTime=-1  ICPrevOutput=DiscIntNeverNeededParam  ICPrevScaledInput=DiscIntNeverNeededParam
  Gain : Gain  Gain=1/10
  Product : Product
  Product7 : Product
  Random Number : RandomNumber  SampleTime=0.1
  Random Number2 : RandomNumber  SampleTime=0.1
  Scope : Scope  NumInputPorts=2
  Scope1 : Scope
  Scope2 : Scope
  Sum : Sum
  brown : Constant  Value=pi
  white : Constant  Value=0.042/180*pi/3
  noise_beta : Outport
  wires:
  Gain/1 -> Sum/2, Scope/2
  Discrete-Time Integrator1/1 -> Gain/1
  Sum/1 -> noise_beta/1, Scope1/1
  brown/1 -> Product7/2
  Product7/1 -> Discrete-Time Integrator1/1, Scope2/1
  Random Number2/1 -> Product7/1
  Random Number/1 -> Product/1
  white/1 -> Product/2
  Product/1 -> Sum/1, Scope/1

== system Detumbling/Subsystem8/Subsystem3/rotation matrix of n ==
  R_B : Inport
  Constant1 : Constant  Value=0
  Demux : Demux  Outputs=3
  Gain{,1,3..4} (4 alike) : Gain  Gain=-1
  Matrix Concatenate : Concatenate  NumInputs=9  ConcatenateDimension=2
  Reshape : Reshape  OutputDimensionality=Customize  OutputDimensions=[3,3]
  Out1 : Outport
  wires:
  Reshape/1 -> Out1/1
  R_B/1 -> Demux/1
  Gain3/1 -> Matrix Concatenate/6
  Demux/3 -> Matrix Concatenate/4, Gain/1
  Demux/2 -> Matrix Concatenate/3, Gain4/1
  Gain/1 -> Matrix Concatenate/2
  Demux/1 -> Matrix Concatenate/8, Gain3/1
  Gain4/1 -> Matrix Concatenate/7
  Matrix Concatenate/1 -> Gain1/1
  Constant1/1 -> Matrix Concatenate/9, Matrix Concatenate/1, Matrix Concatenate/5
  Gain1/1 -> Reshape/1

== system Detumbling/Torque/DRAG_Torque/Force ==
  V_BN : Inport
  Area_vect : Constant  Value=Area_vect
  Constant : Constant  Value=N_b
  Constant1 : Constant  Value=0
  Constant2 : Constant  Value=-0.5*rho*C_d
  Matrix Multiply : Product  Multiplication=Matrix(*)
  Matrix Multiply1 : Product
  Matrix Multiply2 : Product
  Matrix Multiply3 : Product  Multiplication=Matrix(*)
  Matrix Multiply4 : Product  Inputs=3
  Relational Operator : RelationalOperator  Operator=>  OutDataTypeStr=boolean  RndMeth=Simplest  InputSameDT=off
  Square : Math  Operator=square
  Transpose : Math  Operator=transpose
  normalize2 : Subsystem
  Out1 : Outport
  wires:
  Square/1 -> Matrix Multiply4/2
  Matrix Multiply3/1 -> Matrix Multiply4/1
  Matrix Multiply1/1 -> Matrix Multiply2/1
  normalize2/1(vers) -> Transpose/1, Matrix Multiply/2
  Matrix Multiply/1 -> Matrix Multiply1/1, Relational Operator/1
  normalize2/2(norm) -> Square/1
  Constant2/1 -> Matrix Multiply4/3
  Area_vect/1 -> Matrix Multiply2/2
  Constant1/1 -> Relational Operator/2
  Relational Operator/1 -> Matrix Multiply1/2
  Matrix Multiply2/1 -> Matrix Multiply3/1
  Constant/1 -> Matrix Multiply/1
  Transpose/1 -> Matrix Multiply3/2
  Matrix Multiply4/1 -> Out1/1
  V_BN/1 -> normalize2/1(vector)

== system Detumbling/Torque/DRAG_Torque/Sum ==
  In1 : Inport
  Constant8 : Constant  Value=[1;1;1;1;1;1;1;1;1;1]
  Product6 : Product  Multiplication=Matrix(*)
  Transpose1 : Math  Operator=transpose
  Out1 : Outport
  wires:
  Transpose1/1 -> Product6/1
  Product6/1 -> Out1/1
  Constant8/1 -> Product6/2
  In1/1 -> Transpose1/1

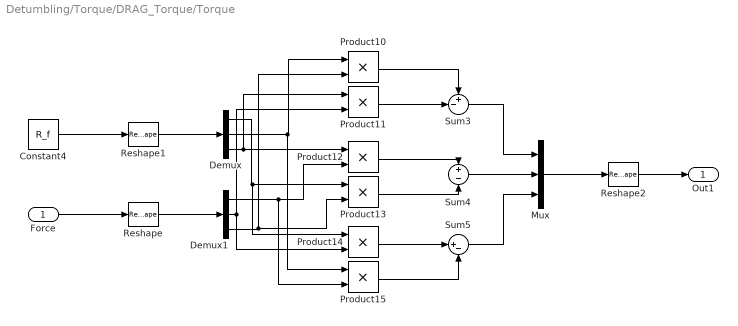
== system Detumbling/Torque/DRAG_Torque/Torque ==
  Force : Inport
  Constant4 : Constant  Value=R_f
  Demux : Demux  Outputs=3
  Demux1 : Demux  Outputs=3
  Mux : Mux  Inputs=3
  Product{10..15} (6 alike) : Product
  Reshape : Reshape  OutputDimensionality=Column vector (2-D)
  Reshape1 : Reshape  OutputDimensionality=Column vector (2-D)
  Reshape2 : Reshape  OutputDimensionality=Customize  OutputDimensions=[n_face,3]
  Sum3 : Sum  Inputs=+-|
  Sum4 : Sum  Inputs=+|-
  Sum5 : Sum  Inputs=|+-
  Out1 : Outport
  wires:
  Product12/1 -> Sum4/1
  Demux1/1 -> Product15/2, Product12/2
  Reshape2/1 -> Out1/1
  Demux/1 -> Product14/1, Product13/1
  Sum5/1 -> Mux/3
  Constant4/1 -> Reshape1/1
  Mux/1 -> Reshape2/1
  Reshape/1 -> Demux1/1
  Demux/3 -> Product12/1, Product11/1
  Demux1/3 -> Product13/2, Product10/2
  Force/1 -> Reshape/1
  Product13/1 -> Sum4/2
  Reshape1/1 -> Demux/1
  Sum3/1 -> Mux/1
  Product11/1 -> Sum3/2
  Demux1/2 -> Product11/2, Product14/2
  Demux/2 -> Product15/1, Product10/1
  Sum4/1 -> Mux/2
  Product14/1 -> Sum5/1
  Product10/1 -> Sum3/1
  Product15/1 -> Sum5/2

== system Detumbling/Torque/DRAG_Torque/V_vect ==
  Theta : Inport
  Constant : Constant  Value=sqrt(mu/p)
  Constant1 : Constant  Value=e
  Constant2 : Constant  Value=0
  Constant3 : Constant  Value=Rot'
  Gain : Gain  Gain=-1
  Mux : Mux  Inputs=3
  Product : Product
  Product1 : Product  Multiplication=Matrix(*)
  Sin : Trigonometry
  Sin1 : Trigonometry  Operator=cos
  Sum : Sum  Inputs=|++
  Out1 : Outport
  wires:
  Constant/1 -> Product/1
  Mux/1 -> Product/2
  Sin/1 -> Gain/1
  Gain/1 -> Mux/1
  Sin1/1 -> Sum/1
  Sum/1 -> Mux/2
  Constant1/1 -> Sum/2
  Theta/1 -> Sin1/1, Sin/1
  Constant2/1 -> Mux/3
  Constant3/1 -> Product1/1
  Product1/1 -> Out1/1
  Product/1 -> Product1/2

== system Detumbling/Torque/GG_Torque/A_BL1 ==
  A_LN : Inport
  A_BN : Inport  Port=2
  Matrix Multiply : Product  Multiplication=Matrix(*)
  Transpose : Math  Operator=transpose
  A_BL : Outport
  wires:
  Transpose/1 -> Matrix Multiply/2
  A_LN/1 -> Transpose/1
  Matrix Multiply/1 -> A_BL/1  "A_BL"
  A_BN/1 -> Matrix Multiply/1

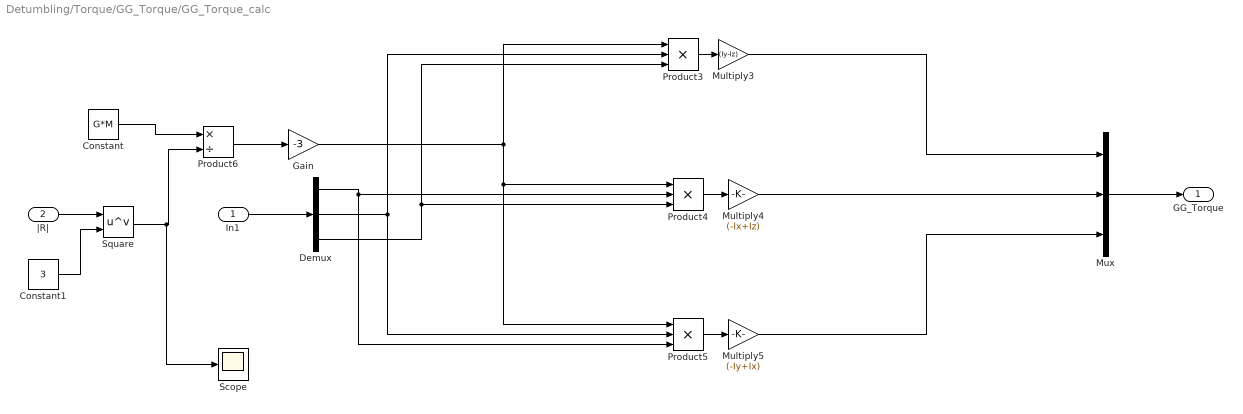
== system Detumbling/Torque/GG_Torque/GG_Torque_calc ==
  In1 : Inport
  |R| : Inport  Port=2
  Constant : Constant  Value=G*M
  Constant1 : Constant  Value=3
  Demux : Demux  Outputs=3
  Gain : Gain  Gain=-3
  Multiply3 : Gain  Gain=(Iy-Iz)
  Multiply4 : Gain  Gain=(-Ix+Iz)
  Multiply5 : Gain  Gain=(-Iy+Ix)
  Mux : Mux  Inputs=3
  Product3 : Product  Inputs=***
  Product4 : Product  Inputs=***
  Product5 : Product  Inputs=***
  Product6 : Product  Inputs=*/
  Scope : Scope
  Square : Math  Operator=pow
  GG_Torque : Outport
  wires:
  Multiply3/1 -> Mux/1
  Mux/1 -> GG_Torque/1
  Multiply4/1 -> Mux/2
  In1/1 -> Demux/1
  Product3/1 -> Multiply3/1
  Gain/1 -> Product5/1, Product4/1, Product3/1
  Demux/2 -> Product3/2, Product5/2
  Demux/3 -> Product3/3, Product4/3
  Product4/1 -> Multiply4/1
  Demux/1 -> Product4/2, Product5/3
  Product5/1 -> Multiply5/1
  Product6/1 -> Gain/1
  Constant/1 -> Product6/1
  |R|/1 -> Square/1
  Constant1/1 -> Square/2
  Square/1 -> Scope/1, Product6/2
  Multiply5/1 -> Mux/3

== system Detumbling/Torque/GG_Torque/Subsystem ==
  A_BL : Inport
  Constant1 : Constant  Value=[1;0;0]
  Matrix Multiply3 : Product  Multiplication=Matrix(*)
  c_vector : Outport
  wires:
  Constant1/1 -> Matrix Multiply3/2
  Matrix Multiply3/1 -> c_vector/1  "c_vector"
  A_BL/1 -> Matrix Multiply3/1

== system Detumbling/Torque/DRAG_Torque/Force/normalize2 ==
  vector : Inport
  Demux : Demux  Outputs=3
  Product : Product  Inputs=*/
  Square : Math  Operator=square
  Square Root : Sqrt
  Square1 : Math  Operator=square
  Square2 : Math  Operator=square
  Sum : Sum  Inputs=+++
  vers : Outport
  norm : Outport  Port=2
  wires:
  Square Root/1 -> norm/1, Product/2
  Demux/3 -> Square2/1
  Square2/1 -> Sum/3
  Square/1 -> Sum/1
  Square1/1 -> Sum/2
  Demux/1 -> Square/1
  Sum/1 -> Square Root/1
  vector/1 -> Product/1, Demux/1
  Demux/2 -> Square1/1
  Product/1 -> vers/1

== matlab function Detumbling/Subsystem5/pseudoinverse ==
  data: u input; y output
function y = fcn(u)
A = u;
% Soluzione con norma minima
x = pinv(A) ;
y = x;

== matlab function Detumbling/Torque/MAG_Torque/MATLAB Function1 ==
  data: r_N input; B_N output; t input; g input; h input
function B_N= fcn(r_N,t,g,h)
[B_N]  = earthmagfield13(r_N/1000, t, g, h, 0, 13);%m->km correction
end
